simulink model "mech_comp"  (R2023a)
settings: Solver=VariableStepAuto  StartTime=0.0  StopTime=5  RelTol=1e-3
libraries: fl_lib x15, nesl_utility x6
settings Model: Creator=ahmad  LastModifiedBy=ahmad

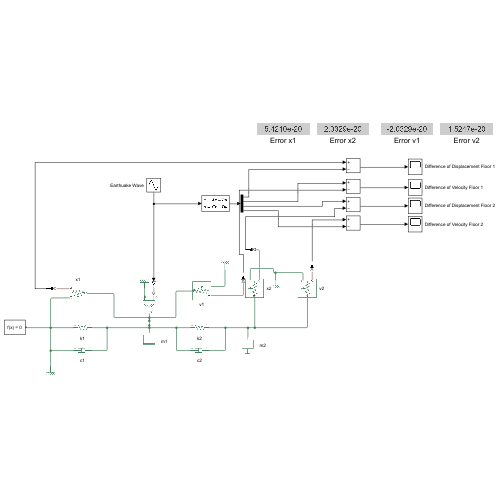
[thumbnail: Simulink's stored preview of the top-level diagram]
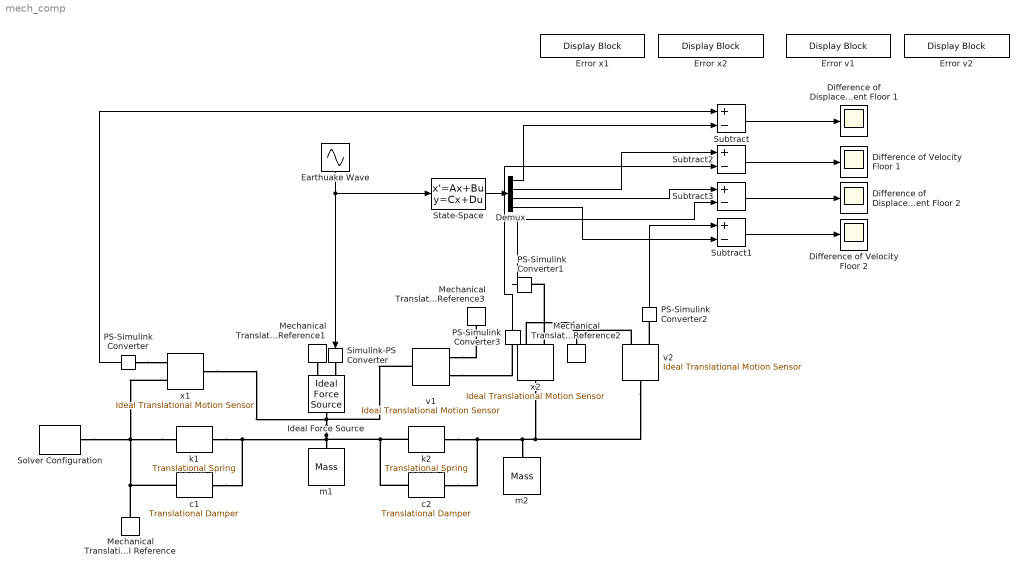
== system mech_comp ==
  Demux : Demux
  Difference of Displacement Floor 1 : Scope
  Difference of Displacement Floor 2 : Scope
  Difference of Velocity Floor 1 : Scope
  Difference of Velocity Floor 2 : Scope
  Earthuake Wave : Sin  Amplitude=5000  Frequency=8*pi  SampleTime=0
  Error v1 : DisplayBlock  LabelPosition=Hide  Transparency=1  Layout=Fill available space
  Error v2 : DisplayBlock  LabelPosition=Hide  Transparency=1  Layout=Fill available space
  Error x1 : DisplayBlock  LabelPosition=Hide  Transparency=1  Layout=Fill available space
  Error x2 : DisplayBlock  LabelPosition=Hide  Transparency=1  Layout=Fill available space
  Ideal Force Source : fl_lib/Mechanical/Mechanical Sources/Ideal Force Source
  Mechanical Translational Reference{,1..3} (4 alike) : fl_lib/Mechanical/Translational Elements/Mechanical Translational Reference
  PS-Simulink Converter{,1..3} (4 alike) : nesl_utility/PS-Simulink Converter  PhysicalDomain=network_engine_domain  SubClassName=ps_output  LeftPortType=input  RightPortType=output  PseudoPeriodic=off  Frequencies=[]  VectorFormat=inherit  Unit=inherit  AffineConversion=off
  Simulink-PS Converter : nesl_utility/Simulink-PS Converter  PhysicalDomain=network_engine_domain  SubClassName=ps_input  LeftPortType=input  RightPortType=output  PseudoPeriodic=off  Frequencies=[]  NoiseDistribution=none  NoiseParameters=[]  Unit=1  AffineConversion=off  FilteringAndDerivatives=provide  SimscapeFilterOrder=1  InputFilterTimeConstant=0.001  UdotUserProvided=0
  Solver Configuration : nesl_utility/Solver Configuration  PhysicalDomain=network_engine_domain  SubClassName=solver  LeftPortType=input  RightPortType=generic  Tones=[]  Harmonics=[]  SimulateNoise=off  Profile=off  UseLocalSampling=off  EnableSwitchedLinearOptims=on  FrequencyDomain=off  UseCCode=off  RelTol=0.001  AbsTol=0.001  MinStep=1e-09  ToWorkspace=off  RevertToSquareIcSolve=off  NumHomotopyIterations=100  PhasorMode=off  PhasorModeNumHarmonics=1  ConsistencySolver=NEWTON_XTOL_AFTER_FTOL  IndexReductionMethod=DerivativeReplacement  DoDC=off  ResidualTolerance=1e-09  ConsistencyTolSource=GLOBAL  ConsistencyAbsTol=0.001  ConsistencyRelTol=0.001  ConsistencyTolFactor=0.001  UseLocalSolver=off  LocalSolverChoice=NE_BACKWARD_EULER_ADVANCER  ResolveIndetEquations=on  FunctionEvalNumThread=1  LocalSolverSampleTime=0.001  DoFixedCost=off  MaxNonlinIter=3  MaxModeIter=2  ComputeImpulses=off  ImpulseIterations=2  LinearAlgebra=auto  LinearAlgebraNumThread=0  EquationFormulation=NE_TIME_EF  DelaysMemoryBudget=1024  AutomaticFiltering=on  FilteringTimeConstant=0.001  PartitionStorageMethod=AS_NEEDED  PartitionMemoryBudget=1024  PartitionMethod=ROBUST
  State-Space : StateSpace  A=[0, 1, 0, 0; -1050, -1500, 50, 500; 0, 0, 0, 1; 1000, 10000, -1000, -10000]  B=[0; 0.00025; 0; 0]  C=[1, 0, 0, 0; 0, 1, 0, 0; 0, 0, 1, 0; 0, 0, 0, 1]  D=[0; 0; 0; 0]  InitialCondition=[0 0 0 0]
  Subtract{,1..3} (4 alike) : Sum  Inputs=+-
  c1 : fl_lib/Mechanical/Translational Elements/Translational Damper  D=4e6 N*s/m  v_specify=on  v_priority=None  v=0 m/s  v_nominal_specify=off  v_nominal_unit=m/s  v_nominal_value=1  f_specify=off  f_priority=None  f=0 N  f_nominal_specify=off  f_nominal_unit=N  f_nominal_value=1
  c2 : fl_lib/Mechanical/Translational Elements/Translational Damper  D=2e6 N*s/m  v_specify=on  v_priority=None  v=0 m/s  v_nominal_specify=off  v_nominal_unit=m/s  v_nominal_value=1  f_specify=off  f_priority=None  f=0 N  f_nominal_specify=off  f_nominal_unit=N  f_nominal_value=1
  k1 : fl_lib/Mechanical/Translational Elements/Translational Spring  spr_rate=4e6 N/m  v_specify=off  v_priority=None  v=0 m/s  v_nominal_specify=off  v_nominal_unit=m/s  v_nominal_value=1  f_specify=off  f_priority=None  f=0 N  f_nominal_specify=off  f_nominal_unit=N  f_nominal_value=1  x_specify=on  x_priority=High  x=0 m  x_nominal_specify=off  x_nominal_unit=m  x_nominal_value=1
  k2 : fl_lib/Mechanical/Translational Elements/Translational Spring  spr_rate=2e5 N/m  v_specify=off  v_priority=None  v=0 m/s  v_nominal_specify=off  v_nominal_unit=m/s  v_nominal_value=1  f_specify=off  f_priority=None  f=0 N  f_nominal_specify=off  f_nominal_unit=N  f_nominal_value=1  x_specify=on  x_priority=High  x=0 m  x_nominal_specify=off  x_nominal_unit=m  x_nominal_value=1
  m1 : fl_lib/Mechanical/Translational Elements/Mass  mass=4000 kg  num_ports=foundation.enum.numPorts2.one  v_specify=off  v_priority=High  v=0 m/s  v_nominal_specify=off  v_nominal_unit=m/s  v_nominal_value=1  f_specify=off  f_priority=None  f=0 N  f_nominal_specify=off  f_nominal_unit=N  f_nominal_value=1
  m2 : fl_lib/Mechanical/Translational Elements/Mass  mass=200 kg  num_ports=foundation.enum.numPorts2.one  v_specify=off  v_priority=High  v=0 m/s  v_nominal_specify=off  v_nominal_unit=m/s  v_nominal_value=1  f_specify=off  f_priority=None  f=0 N  f_nominal_specify=off  f_nominal_unit=N  f_nominal_value=1
  v1 : fl_lib/Mechanical/Mechanical Sensors/Ideal Translational Motion Sensor  reference=foundation.enum.MeasurementReference.difference  acceleration_port=false  velocity_port=true  position_port=false  offset=0 m
      settings: InternalSimscapePortConfiguration="{\"Bottom\":[],\"Left\":[{\"id\":\"R\",\"label\":\"R\",\"type\":\"foundation.mechanical.translational.translational\"}],\"Right\":[{\"id\":\"C\",\"label\":\"C\",\"type\":\"foundation.mechanical.translational.translational\"},{\"id\":\"V\",\"label\":\"V\",\"type\":\"output\"}],\"Top\":[]}"
  v2 : fl_lib/Mechanical/Mechanical Sensors/Ideal Translational Motion Sensor  reference=foundation.enum.MeasurementReference.difference  acceleration_port=false  velocity_port=true  position_port=false  offset=0 m
      settings: InternalSimscapePortConfiguration="{\"Bottom\":[],\"Left\":[{\"id\":\"R\",\"label\":\"R\",\"type\":\"foundation.mechanical.translational.translational\"}],\"Right\":[{\"id\":\"C\",\"label\":\"C\",\"type\":\"foundation.mechanical.translational.translational\"},{\"id\":\"V\",\"label\":\"V\",\"type\":\"output\"}],\"Top\":[]}"
  x1 : fl_lib/Mechanical/Mechanical Sensors/Ideal Translational Motion Sensor  reference=foundation.enum.MeasurementReference.difference  acceleration_port=false  velocity_port=false  position_port=true  offset=0 m
      settings: InternalSimscapePortConfiguration="{\"Bottom\":[],\"Left\":[{\"id\":\"R\",\"label\":\"R\",\"type\":\"foundation.mechanical.translational.translational\"}],\"Right\":[{\"id\":\"C\",\"label\":\"C\",\"type\":\"foundation.mechanical.translational.translational\"},{\"id\":\"P\",\"label\":\"P\",\"type\":\"output\"}],\"Top\":[]}"
  x2 : fl_lib/Mechanical/Mechanical Sensors/Ideal Translational Motion Sensor  reference=foundation.enum.MeasurementReference.difference  acceleration_port=false  velocity_port=false  position_port=true  offset=0 m
      settings: InternalSimscapePortConfiguration="{\"Bottom\":[],\"Left\":[{\"id\":\"R\",\"label\":\"R\",\"type\":\"foundation.mechanical.translational.translational\"}],\"Right\":[{\"id\":\"C\",\"label\":\"C\",\"type\":\"foundation.mechanical.translational.translational\"},{\"id\":\"P\",\"label\":\"P\",\"type\":\"output\"}],\"Top\":[]}"
  wires:
  State-Space/1 -> Demux/1
  Earthuake Wave/1 -> State-Space/1, Simulink-PS Converter/1
  PS-Simulink Converter/1 -> Subtract/1
  PS-Simulink Converter2/1 -> Subtract1/1
  Demux/1 -> Subtract/2
  Demux/4 -> Subtract1/2
  Subtract1/1 -> Difference of Velocity Floor 2/1
  Subtract/1 -> Difference of Displacement Floor 1/1
  Demux/2 -> Subtract2/1
  Subtract2/1 -> Difference of Velocity Floor 1/1
  PS-Simulink Converter3/1 -> Subtract2/2
  Demux/3 -> Subtract3/1
  PS-Simulink Converter1/1 -> Subtract3/2
  Subtract3/1 -> Difference of Displacement Floor 2/1
  connections:
  x2/LConn1 -- k2/RConn1 -- c2/RConn1 -- m2/LConn1 -- v2/LConn1
  x1/LConn1 -- k1/RConn1 -- c1/RConn1 -- c2/LConn1 -- k2/LConn1 -- m1/LConn1 -- Ideal Force Source/LConn1 -- v1/LConn1
  Mechanical Translational Reference2/LConn1 -- x2/RConn1 -- v2/RConn1
  k1/LConn1 -- Mechanical Translational Reference/LConn1 -- c1/LConn1 -- Solver Configuration/RConn1 -- x1/RConn1
  x2/RConn2 -- PS-Simulink Converter1/LConn1
  v2/RConn2 -- PS-Simulink Converter2/LConn1
  Simulink-PS Converter/RConn1 -- Ideal Force Source/RConn1
  v1/RConn2 -- PS-Simulink Converter3/LConn1
  PS-Simulink Converter/LConn1 -- x1/RConn2
  Mechanical Translational Reference1/LConn1 -- Ideal Force Source/RConn2
  v1/RConn1 -- Mechanical Translational Reference3/LConn1
